simulink model "fi_sb2"  (R2026a)
settings: Solver=VariableStepAuto  StopTime=24.0
libraries: deeplib x1
settings Model: Creator=ldy  LastModifiedBy=harry_31916

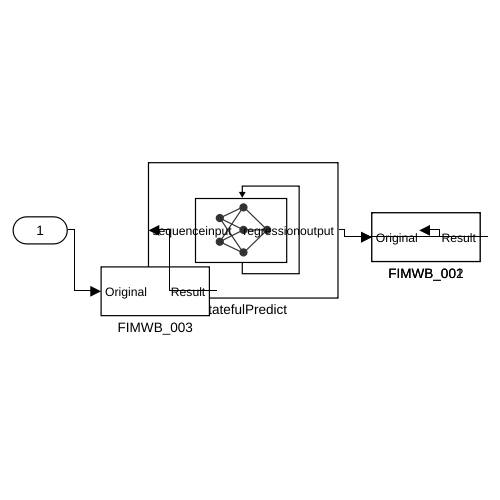
[thumbnail: Simulink's stored preview of the top-level diagram]
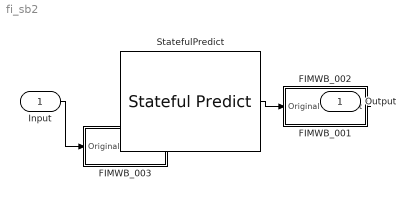
== system fi_sb2 ==
  Input : Inport
  FIMWB_001 : Subsystem  Tag=fimwb.fault.1
  FIMWB_002 : Subsystem  Tag=fimwb.fault.2
  FIMWB_003 : Subsystem  Tag=fimwb.fault.3
  StatefulPredict : deeplib/Stateful Predict  Network=Network from MAT-file  NetworkFunction=untitled  NetworkFilePath=phi2_m1_vr01_k2_2.mat  SimulateUsing=Auto mode  InputDataFormats={'',''}  SampleTime=1  ForceInterpretedSim=off  EnableDLNetwork=on  LastKnownNetworkFilePath=''  LastKnownNetworkTimeStamp=''
  Output : Outport
  wires:
  StatefulPredict/1 -> FIMWB_001/1(Original)
  FIMWB_001/1(Result) -> FIMWB_002/1(Original)
  FIMWB_002/1(Result) -> Output/1
  Input/1 -> FIMWB_003/1(Original)
  FIMWB_003/1(Result) -> StatefulPredict/1

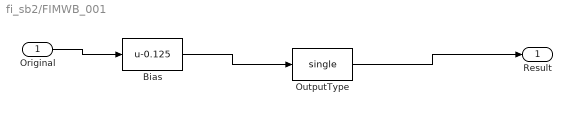
== system fi_sb2/FIMWB_001 ==
  Original : Inport
  Bias : Bias  Bias=-0.125  SaturateOnIntegerOverflow=off
  OutputType : DataTypeConversion  OutDataTypeStr=single  RndMeth=Round
  Result : Outport
  wires:
  Original/1 -> Bias/1
  Bias/1 -> OutputType/1
  OutputType/1 -> Result/1

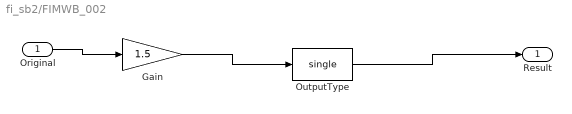
== system fi_sb2/FIMWB_002 ==
  Original : Inport
  Gain : Gain  Gain=1.5  OutDataTypeStr=Inherit: Same as input
  OutputType : DataTypeConversion  OutDataTypeStr=single  RndMeth=Round
  Result : Outport
  wires:
  Original/1 -> Gain/1
  Gain/1 -> OutputType/1
  OutputType/1 -> Result/1

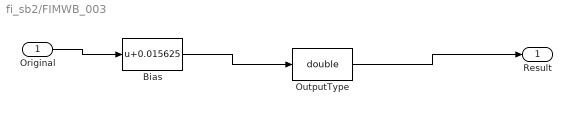
== system fi_sb2/FIMWB_003 ==
  Original : Inport
  Bias : Bias  Bias=0.015625  SaturateOnIntegerOverflow=off
  OutputType : DataTypeConversion  OutDataTypeStr=double  RndMeth=Round
  Result : Outport
  wires:
  Original/1 -> Bias/1
  Bias/1 -> OutputType/1
  OutputType/1 -> Result/1
